simulink model "lab1"  (R2023a)
settings: Solver=VariableStepAuto  StartTime=0.0  StopTime=10.0  MaxStep=0.01  RelTol=1e-3
settings Model: SnapshotBufferSize=100  Creator=Admin  LastModifiedBy=Admin

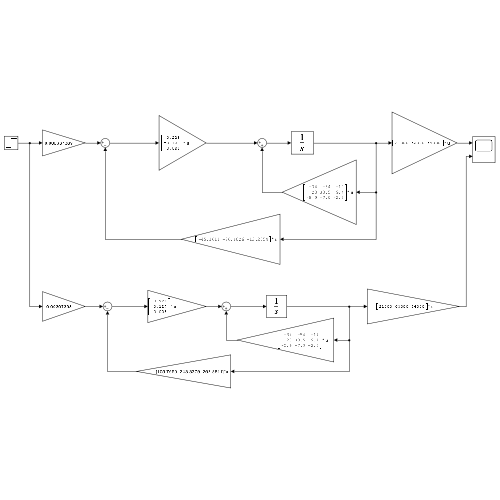
[thumbnail: Simulink's stored preview of the top-level diagram]
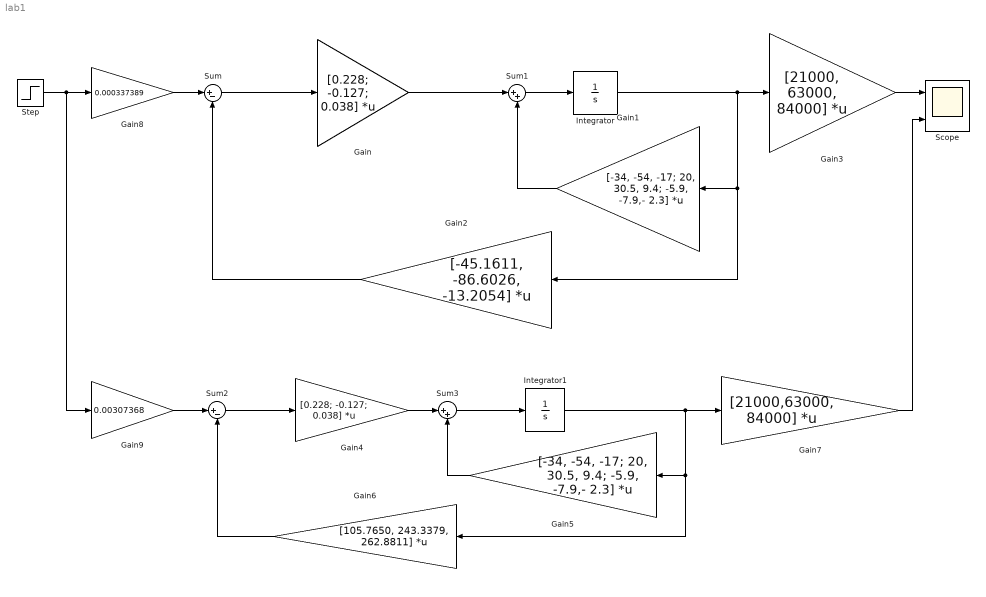
== system lab1 ==
  Gain : Gain  Gain=[0.228; -0.127; 0.038]  Multiplication=Matrix(K*u)
  Gain1 : Gain  Gain=[-34, -54, -17; 20, 30.5, 9.4; -5.9, -7.9,- 2.3]  Multiplication=Matrix(K*u)
  Gain2 : Gain  Gain=[-45.1611, -86.6026, -13.2054]  Multiplication=Matrix(K*u)
  Gain3 : Gain  Gain=[21000, 63000, 84000]  Multiplication=Matrix(K*u)
  Gain4 : Gain  Gain=[0.228; -0.127; 0.038]  Multiplication=Matrix(K*u)
  Gain5 : Gain  Gain=[-34, -54, -17; 20, 30.5, 9.4; -5.9, -7.9,- 2.3]  Multiplication=Matrix(K*u)
  Gain6 : Gain  Gain=[105.7650, 243.3379, 262.8811]  Multiplication=Matrix(K*u)
  Gain7 : Gain  Gain=[21000,63000, 84000]  Multiplication=Matrix(K*u)
  Gain8 : Gain  Gain=0.000337389
  Gain9 : Gain  Gain=0.00307368
  Integrator : Integrator
  Integrator1 : Integrator
  Scope : Scope  NumInputPorts=2
  Step : Step  Time=0  SampleTime=0
  Sum : Sum  Inputs=|+-
  Sum1 : Sum  Inputs=|++
  Sum2 : Sum  Inputs=|+-
  Sum3 : Sum  Inputs=|++
  wires:
  Sum/1 -> Gain/1
  Sum1/1 -> Integrator/1
  Gain1/1 -> Sum1/2
  Integrator/1 -> Gain2/1, Gain1/1, Gain3/1
  Gain/1 -> Sum1/1
  Gain2/1 -> Sum/2
  Gain3/1 -> Scope/1
  Gain4/1 -> Sum3/1
  Sum2/1 -> Gain4/1
  Gain7/1 -> Scope/2
  Integrator1/1 -> Gain6/1, Gain5/1, Gain7/1
  Gain5/1 -> Sum3/2
  Sum3/1 -> Integrator1/1
  Step/1 -> Gain9/1, Gain8/1
  Gain6/1 -> Sum2/2
  Gain8/1 -> Sum/1
  Gain9/1 -> Sum2/1
